simulink model "laser_udp_test"  (R2025b)
settings: Solver=FixedStepDiscrete  StartTime=0.0  StopTime=inf  FixedStep=0.05  RelTol=1e-3  EnableMultiTasking=on
libraries: raspberrypiBasiclib x1, raspberrypiNetworklib x1
settings Model: ExtModeTrigDuration=2  Creator=jeets  LastModifiedBy=jeets
settings SolverCC: PositivePriorityOrder=on
settings OptimizationCC: EnhancedBackFolding=on  PassReuseOutputArgsAs=Individual arguments  ZeroExternalMemoryAtStartup=off  ZeroInternalMemoryAtStartup=off  MaxStackSize=200000  OptimizeBlockOrder=speed  DifferentSizesBufferReuse=on  OptimizationCustomize=off  EfficientTunableParamExpr=on
settings DebuggingCC: ParameterTunabilityLossMsg=error
settings HardwareCC: ProdBitPerPointer=32.0  ProdBitPerSizeT=32.0  ProdBitPerPtrDiffT=32.0  ProdLargestAtomicInteger=Long  ProdLargestAtomicFloat=Double  ProdWordSize=32.0  ProdLongLongMode=on  ProdHWDeviceType=ARM Compatible->ARM Cortex-A (32-bit)
settings RTWCC: SystemTargetFile=ert.tlc  HardwareBoard=Raspberry Pi  TLCOptions="-aInlineSetEventsForThisBaseRateFcn=TLC_FALSE -aSuppressMultiTaskScheduler=TLC_FALSE  -aRateBasedStepFcn=0"  TemplateMakefile=ert_default_tmf  Toolchain=GNU GCC Embedded Linux  BuildConfiguration=Faster Runs  Description=Embedded Coder
settings CodeAppCC: ForceParamTrailComments=on  IgnoreCustomStorageClasses=off  OperatorAnnotations=on  SimulinkDataObjDesc=on  SFDataObjDesc=on  InsertBlockDesc=on
settings ERTTargetCC: ExtModeTransport=2.0  ExtModeStaticAlloc=on  ExtModeMexFile=ext_xcp  ExtModeIntrfLevel=Level2 - Open  InlinedParameterPlacement=Hierarchical  CodeReplacementLibrary=ARM Cortex-A CMSIS  SupportVariableSizeSignals=on

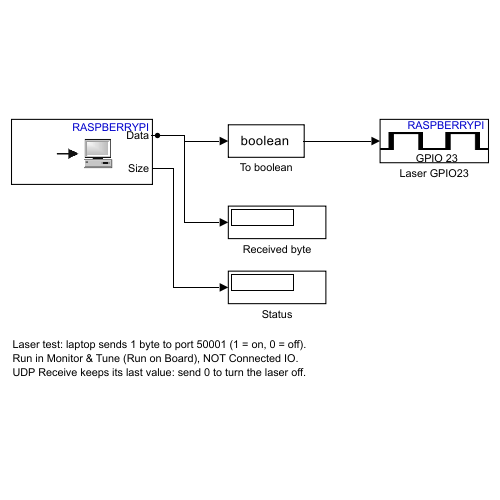
[thumbnail: Simulink's stored preview of the top-level diagram]
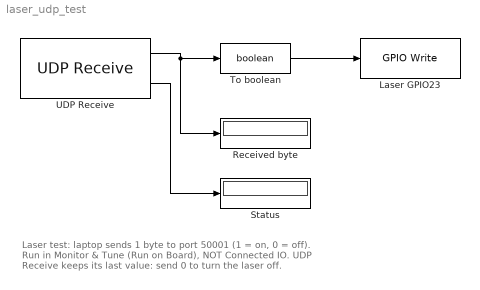
== system laser_udp_test ==
  note: Laser test: laptop sends 1 byte to port 50001 (1 = on, 0 = off).
      | Run in Monitor & Tune (Run on Board), NOT Connected IO.
      | UDP Receive keeps its last value: send 0 to turn the laser off.
  Laser GPIO23 : raspberrypiBasiclib/GPIO Write  BoardProperty=Pi 4 Model B  gpio=23  blockPlatform=Raspberry Pi  PinNumber=17  board=[]  direction=[]
  Received byte : Display
  Status : Display
  To boolean : DataTypeConversion  OutDataTypeStr=boolean  SaturateOnIntegerOverflow=off  RndMeth=Floor
  UDP Receive : raspberrypiNetworklib/UDP Receive  localURL='0.0.0.0'  localPort=50001  remoteURL='0.0.0.0'  remotePort=-1  recvBufferSize=8192  signalDatatype=uint8  dims=1  isVarSize=off  showBlockingTime=off  blockingTime=0  sampletime=0.05  blockPlatform=Raspberry Pi
  wires:
  UDP Receive/1 -> To boolean/1, Received byte/1
  To boolean/1 -> Laser GPIO23/1
  UDP Receive/2 -> Status/1
